simulink model "Proyecto1"  (R2023a)
settings: Solver=ode15s  StartTime=0.0  StopTime=12  MaxStep=0.0001  RelTol=1e-7  AbsTol=1e-9
libraries: fl_lib x22, nesl_utility x6, slpidlib x1
settings Model: Creator=ediel  LastModifiedBy=Chulis
settings SolverCC: AlgebraicLoopSolver=TrustRegion
settings DataIOCC: SaveOutput=off  SignalLogging=off  DSMLogging=off  ReturnWorkspaceOutputs=off  TimeSaveName=t
settings DebuggingCC: AlgebraicLoopMsg=none  ArtificialAlgebraicLoopMsg=none  MaxConsecutiveZCsMsg=none  UnconnectedInputMsg=warning  UnconnectedOutputMsg=warning  UnconnectedLineMsg=warning  ModelReferenceExtraNoncontSigs=none  OperatingPointInterfaceChecksumMismatchMsg=none
settings ModelReferenceCC: EnableRefExpFcnMdlSchedulingChecks=on
settings RTWCC: DLArmComputeVersion=19.05

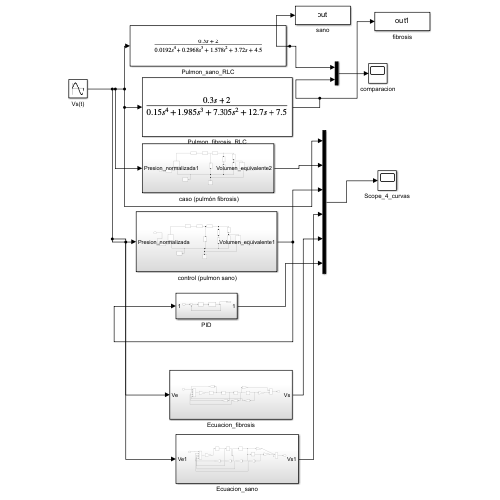
[thumbnail: Simulink's stored preview of the top-level diagram]
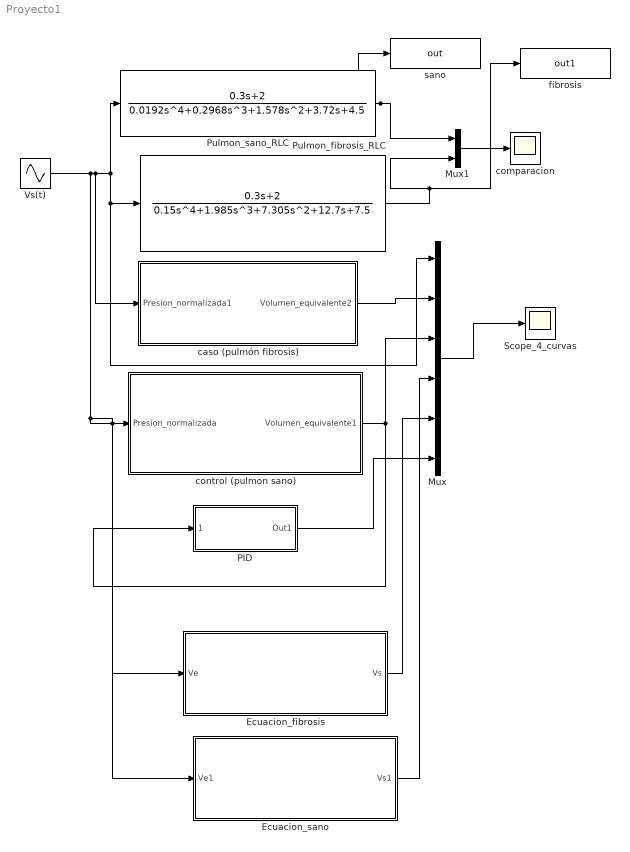
== system Proyecto1 ==
  " caso (pulmón fibrosis)" : Subsystem
  " control (pulmon sano)" : Subsystem
  Ecuacion_fibrosis : Subsystem
  Ecuacion_sano : Subsystem
  Mux : Mux  Inputs=6
  Mux1 : Mux  Inputs=2
  PID : Subsystem
  Pulmon_fibrosis_RLC : TransferFcn  Numerator=[0.3 2]  Denominator=[0.15,1.985,7.305,12.7,7.5]
  Pulmon_sano_RLC : TransferFcn  Numerator=[0.3 2]  Denominator=[0.0192,0.2968,1.578,3.72,4.5]
  Scope_4_curvas : Scope
  Vs(t) : Sin  Amplitude=0.5  Bias=0.5  Frequency=pi/2  Phase=-pi/2  SampleTime=0
  comparacion : Scope
  fibrosis : ToWorkspace  VariableName=out1  SaveFormat=Timeseries  SampleTime=-1
  sano : ToWorkspace  VariableName=out  SaveFormat=Timeseries  SampleTime=-1
  wires:
  Vs(t)/1 -> Ecuacion_sano/1(Ve1), Ecuacion_fibrosis/1(Ve), " control (pulmon sano)"/1(Presion_normalizada), Mux/1, Pulmon_fibrosis_RLC/1, Pulmon_sano_RLC/1, " caso (pulmón fibrosis)"/1(Presion_normalizada1)
  Pulmon_fibrosis_RLC/1 -> Mux1/2, fibrosis/1
  Pulmon_sano_RLC/1 -> Mux1/1, sano/1
  Mux/1 -> Scope_4_curvas/1
  " control (pulmon sano)"/1(Volumen_equivalente1) -> PID/1(1), Mux/3
  Mux1/1 -> comparacion/1
  " caso (pulmón fibrosis)"/1(Volumen_equivalente2) -> Mux/2
  PID/1(Out1) -> Mux/6
  Ecuacion_fibrosis/1(Vs) -> Mux/5
  Ecuacion_sano/1(Vs1) -> Mux/4

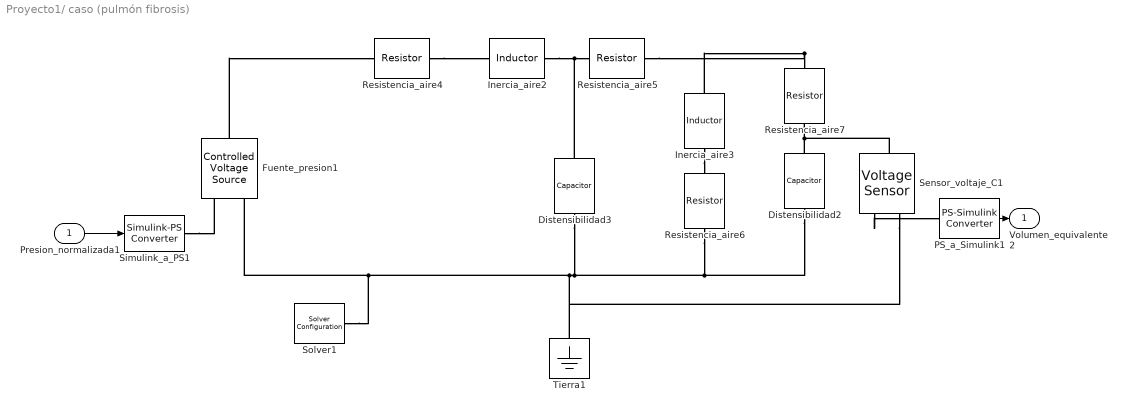
== system Proyecto1/ caso (pulmón fibrosis) ==
  Presion_normalizada1 : Inport
  Distensibilidad2 : fl_lib/Electrical/Electrical Elements/Capacitor  c=0.4 F  r=1e-6 Ohm  g=0 1/Ohm  i_specify=off  i_priority=None  i=0 A  i_nominal_specify=off  i_nominal_unit=A  i_nominal_value=1  v_specify=off  v_priority=None  v=0 V  v_nominal_specify=off  v_nominal_unit=V  v_nominal_value=1  vc_specify=off  vc_priority=High  vc=0 V  vc_nominal_specify=off  vc_nominal_unit=V  vc_nominal_value=1
  Distensibilidad3 : fl_lib/Electrical/Electrical Elements/Capacitor  c=0.5 F  r=1e-6 Ohm  g=0 1/Ohm  i_specify=off  i_priority=None  i=0 A  i_nominal_specify=off  i_nominal_unit=A  i_nominal_value=1  v_specify=off  v_priority=None  v=0 V  v_nominal_specify=off  v_nominal_unit=V  v_nominal_value=1  vc_specify=off  vc_priority=High  vc=0 V  vc_nominal_specify=off  vc_nominal_unit=V  vc_nominal_value=1
  Fuente_presion1 : fl_lib/Electrical/Electrical Sources/Controlled Voltage Source
  Inercia_aire2 : fl_lib/Electrical/Electrical Elements/Inductor  l=0.5 H  r=0.5 Ohm  g=1e-9 1/Ohm  i_specify=off  i_priority=None  i=0 A  i_nominal_specify=off  i_nominal_unit=A  i_nominal_value=1  v_specify=off  v_priority=None  v=0 V  v_nominal_specify=off  v_nominal_unit=V  v_nominal_value=1  i_L_specify=off  i_L_priority=High  i_L=0 A  i_L_nominal_specify=off  i_L_nominal_unit=A  i_L_nominal_value=1
  Inercia_aire3 : fl_lib/Electrical/Electrical Elements/Inductor  l=0.3 H  r=0 Ohm  g=1e-9 1/Ohm  i_specify=off  i_priority=None  i=0 A  i_nominal_specify=off  i_nominal_unit=A  i_nominal_value=1  v_specify=off  v_priority=None  v=0 V  v_nominal_specify=off  v_nominal_unit=V  v_nominal_value=1  i_L_specify=off  i_L_priority=High  i_L=0 A  i_L_nominal_specify=off  i_L_nominal_unit=A  i_L_nominal_value=1
  PS_a_Simulink1 : nesl_utility/PS-Simulink Converter  PhysicalDomain=network_engine_domain  SubClassName=ps_output  LeftPortType=input  RightPortType=output  PseudoPeriodic=off  Frequencies=[]  VectorFormat=1-D array  Unit=V  AffineConversion=off
  Resistencia_aire4 : fl_lib/Electrical/Electrical Elements/Resistor  R=1 Ohm  i_specify=off  i_priority=None  i=0 A  i_nominal_specify=off  i_nominal_unit=A  i_nominal_value=1  v_specify=off  v_priority=None  v=0 V  v_nominal_specify=off  v_nominal_unit=V  v_nominal_value=1
  Resistencia_aire5 : fl_lib/Electrical/Electrical Elements/Resistor  R=4 Ohm  i_specify=off  i_priority=None  i=0 A  i_nominal_specify=off  i_nominal_unit=A  i_nominal_value=1  v_specify=off  v_priority=None  v=0 V  v_nominal_specify=off  v_nominal_unit=V  v_nominal_value=1
  Resistencia_aire6 : fl_lib/Electrical/Electrical Elements/Resistor  R=2 Ohm  i_specify=off  i_priority=None  i=0 A  i_nominal_specify=off  i_nominal_unit=A  i_nominal_value=1  v_specify=off  v_priority=None  v=0 V  v_nominal_specify=off  v_nominal_unit=V  v_nominal_value=1
  Resistencia_aire7 : fl_lib/Electrical/Electrical Elements/Resistor  R=1 Ohm  i_specify=off  i_priority=None  i=0 A  i_nominal_specify=off  i_nominal_unit=A  i_nominal_value=1  v_specify=off  v_priority=None  v=0 V  v_nominal_specify=off  v_nominal_unit=V  v_nominal_value=1
  Sensor_voltaje_C1 : fl_lib/Electrical/Electrical Sensors/Voltage Sensor
  Simulink_a_PS1 : nesl_utility/Simulink-PS Converter  PhysicalDomain=network_engine_domain  SubClassName=ps_input  LeftPortType=input  RightPortType=output  PseudoPeriodic=off  Frequencies=[]  NoiseDistribution=none  NoiseParameters=[]  Unit=V  AffineConversion=off  FilteringAndDerivatives=provide  SimscapeFilterOrder=1  InputFilterTimeConstant=0.001  UdotUserProvided=0
  Solver1 : nesl_utility/Solver Configuration  PhysicalDomain=network_engine_domain  SubClassName=solver  LeftPortType=input  RightPortType=generic  Tones=[]  Harmonics=[]  SimulateNoise=off  Profile=off  UseLocalSampling=off  EnableSwitchedLinearOptims=on  FrequencyDomain=off  UseCCode=off  RelTol=0.001  AbsTol=1e-06  MinStep=1e-09  ToWorkspace=off  RevertToSquareIcSolve=off  NumHomotopyIterations=100  PhasorMode=off  PhasorModeNumHarmonics=1  ConsistencySolver=NEWTON_FTOL  IndexReductionMethod=DerivativeReplacement  DoDC=off  ResidualTolerance=1e-09  ConsistencyTolSource=GLOBAL  ConsistencyAbsTol=0.001  ConsistencyRelTol=0.001  ConsistencyTolFactor=0.001  UseLocalSolver=off  LocalSolverChoice=NE_BACKWARD_EULER_ADVANCER  ResolveIndetEquations=on  FunctionEvalNumThread=1  LocalSolverSampleTime=0.001  DoFixedCost=off  MaxNonlinIter=3  MaxModeIter=2  ComputeImpulses=off  ImpulseIterations=2  LinearAlgebra=auto  LinearAlgebraNumThread=0  EquationFormulation=NE_TIME_EF  DelaysMemoryBudget=1024  AutomaticFiltering=on  FilteringTimeConstant=0.001  PartitionStorageMethod=AS_NEEDED  PartitionMemoryBudget=1024  PartitionMethod=ROBUST
  Tierra1 : fl_lib/Electrical/Electrical Elements/Electrical Reference
  Volumen_equivalente2 : Outport
  wires:
  PS_a_Simulink1/1 -> Volumen_equivalente2/1
  Presion_normalizada1/1 -> Simulink_a_PS1/1
  connections:
  Resistencia_aire5/LConn1 -- Distensibilidad3/LConn1 -- Inercia_aire2/RConn1
  Resistencia_aire7/LConn1 -- Resistencia_aire5/RConn1 -- Inercia_aire3/LConn1
  Resistencia_aire6/RConn1 -- Sensor_voltaje_C1/RConn2 -- Tierra1/LConn1 -- Solver1/RConn1 -- Fuente_presion1/RConn2 -- Distensibilidad3/RConn1 -- Distensibilidad2/RConn1
  Fuente_presion1/LConn1 -- Resistencia_aire4/LConn1
  Resistencia_aire4/RConn1 -- Inercia_aire2/LConn1
  Inercia_aire3/RConn1 -- Resistencia_aire6/LConn1
  Distensibilidad2/LConn1 -- Sensor_voltaje_C1/LConn1 -- Resistencia_aire7/RConn1
  Simulink_a_PS1/RConn1 -- Fuente_presion1/RConn1
  Sensor_voltaje_C1/RConn1 -- PS_a_Simulink1/LConn1

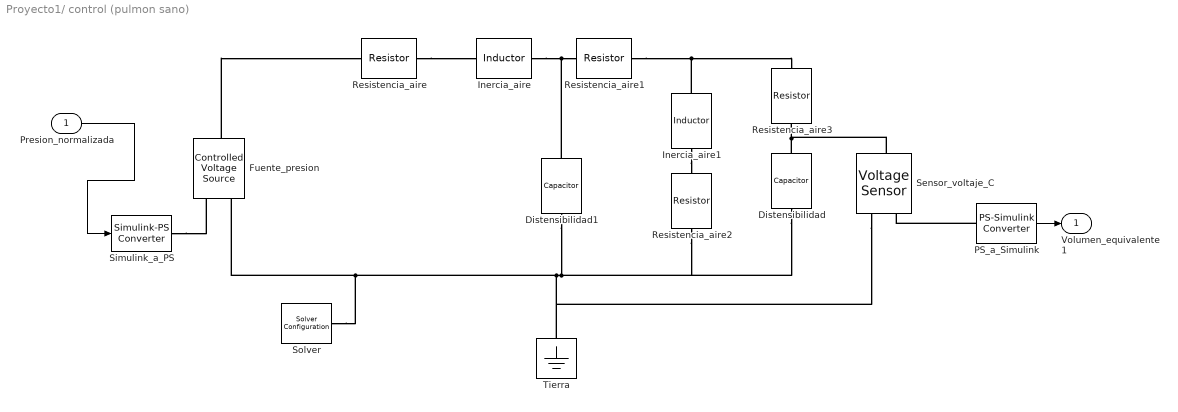
== system Proyecto1/ control (pulmon sano) ==
  Presion_normalizada : Inport
  Distensibilidad : fl_lib/Electrical/Electrical Elements/Capacitor  c=0.16 F  r=1e-6 Ohm  g=0 1/Ohm  i_specify=off  i_priority=None  i=0 A  i_nominal_specify=off  i_nominal_unit=A  i_nominal_value=1  v_specify=off  v_priority=None  v=0 V  v_nominal_specify=off  v_nominal_unit=V  v_nominal_value=1  vc_specify=off  vc_priority=High  vc=0 V  vc_nominal_specify=off  vc_nominal_unit=V  vc_nominal_value=1
  Distensibilidad1 : fl_lib/Electrical/Electrical Elements/Capacitor  c=0.2 F  r=1e-6 Ohm  g=0 1/Ohm  i_specify=off  i_priority=None  i=0 A  i_nominal_specify=off  i_nominal_unit=A  i_nominal_value=1  v_specify=off  v_priority=None  v=0 V  v_nominal_specify=off  v_nominal_unit=V  v_nominal_value=1  vc_specify=off  vc_priority=High  vc=0 V  vc_nominal_specify=off  vc_nominal_unit=V  vc_nominal_value=1
  Fuente_presion : fl_lib/Electrical/Electrical Sources/Controlled Voltage Source
  Inercia_aire : fl_lib/Electrical/Electrical Elements/Inductor  l=1 H  r=0.5 Ohm  g=1e-9 1/Ohm  i_specify=off  i_priority=None  i=0 A  i_nominal_specify=off  i_nominal_unit=A  i_nominal_value=1  v_specify=off  v_priority=None  v=0 V  v_nominal_specify=off  v_nominal_unit=V  v_nominal_value=1  i_L_specify=off  i_L_priority=High  i_L=0 A  i_L_nominal_specify=off  i_L_nominal_unit=A  i_L_nominal_value=1
  Inercia_aire1 : fl_lib/Electrical/Electrical Elements/Inductor  l=0.3 H  r=0 Ohm  g=1e-9 1/Ohm  i_specify=off  i_priority=None  i=0 A  i_nominal_specify=off  i_nominal_unit=A  i_nominal_value=1  v_specify=off  v_priority=None  v=0 V  v_nominal_specify=off  v_nominal_unit=V  v_nominal_value=1  i_L_specify=off  i_L_priority=High  i_L=0 A  i_L_nominal_specify=off  i_L_nominal_unit=A  i_L_nominal_value=1
  PS_a_Simulink : nesl_utility/PS-Simulink Converter  PhysicalDomain=network_engine_domain  SubClassName=ps_output  LeftPortType=input  RightPortType=output  PseudoPeriodic=off  Frequencies=[]  VectorFormat=1-D array  Unit=V  AffineConversion=off
  Resistencia_aire : fl_lib/Electrical/Electrical Elements/Resistor  R=1 Ohm  i_specify=off  i_priority=None  i=0 A  i_nominal_specify=off  i_nominal_unit=A  i_nominal_value=1  v_specify=off  v_priority=None  v=0 V  v_nominal_specify=off  v_nominal_unit=V  v_nominal_value=1
  Resistencia_aire1 : fl_lib/Electrical/Electrical Elements/Resistor  R=1 Ohm  i_specify=off  i_priority=None  i=0 A  i_nominal_specify=off  i_nominal_unit=A  i_nominal_value=1  v_specify=off  v_priority=None  v=0 V  v_nominal_specify=off  v_nominal_unit=V  v_nominal_value=1
  Resistencia_aire2 : fl_lib/Electrical/Electrical Elements/Resistor  R=2 Ohm  i_specify=off  i_priority=None  i=0 A  i_nominal_specify=off  i_nominal_unit=A  i_nominal_value=1  v_specify=off  v_priority=None  v=0 V  v_nominal_specify=off  v_nominal_unit=V  v_nominal_value=1
  Resistencia_aire3 : fl_lib/Electrical/Electrical Elements/Resistor  R=1 Ohm  i_specify=off  i_priority=None  i=0 A  i_nominal_specify=off  i_nominal_unit=A  i_nominal_value=1  v_specify=off  v_priority=None  v=0 V  v_nominal_specify=off  v_nominal_unit=V  v_nominal_value=1
  Sensor_voltaje_C : fl_lib/Electrical/Electrical Sensors/Voltage Sensor
  Simulink_a_PS : nesl_utility/Simulink-PS Converter  PhysicalDomain=network_engine_domain  SubClassName=ps_input  LeftPortType=input  RightPortType=output  PseudoPeriodic=off  Frequencies=[]  NoiseDistribution=none  NoiseParameters=[]  Unit=V  AffineConversion=off  FilteringAndDerivatives=provide  SimscapeFilterOrder=1  InputFilterTimeConstant=0.001  UdotUserProvided=0
  Solver : nesl_utility/Solver Configuration  PhysicalDomain=network_engine_domain  SubClassName=solver  LeftPortType=input  RightPortType=generic  Tones=[]  Harmonics=[]  SimulateNoise=off  Profile=off  UseLocalSampling=off  EnableSwitchedLinearOptims=on  FrequencyDomain=off  UseCCode=off  RelTol=0.001  AbsTol=1e-06  MinStep=1e-09  ToWorkspace=off  RevertToSquareIcSolve=off  NumHomotopyIterations=100  PhasorMode=off  PhasorModeNumHarmonics=1  ConsistencySolver=NEWTON_FTOL  IndexReductionMethod=DerivativeReplacement  DoDC=off  ResidualTolerance=1e-09  ConsistencyTolSource=GLOBAL  ConsistencyAbsTol=0.001  ConsistencyRelTol=0.001  ConsistencyTolFactor=0.001  UseLocalSolver=off  LocalSolverChoice=NE_BACKWARD_EULER_ADVANCER  ResolveIndetEquations=on  FunctionEvalNumThread=1  LocalSolverSampleTime=0.001  DoFixedCost=off  MaxNonlinIter=3  MaxModeIter=2  ComputeImpulses=off  ImpulseIterations=2  LinearAlgebra=auto  LinearAlgebraNumThread=0  EquationFormulation=NE_TIME_EF  DelaysMemoryBudget=1024  AutomaticFiltering=on  FilteringTimeConstant=0.001  PartitionStorageMethod=AS_NEEDED  PartitionMemoryBudget=1024  PartitionMethod=ROBUST
  Tierra : fl_lib/Electrical/Electrical Elements/Electrical Reference
  Volumen_equivalente1 : Outport
  wires:
  Presion_normalizada/1 -> Simulink_a_PS/1
  PS_a_Simulink/1 -> Volumen_equivalente1/1
  connections:
  Solver/RConn1 -- Sensor_voltaje_C/RConn2 -- Tierra/LConn1 -- Distensibilidad/RConn1 -- Resistencia_aire2/RConn1 -- Distensibilidad1/RConn1 -- Fuente_presion/RConn2
  Resistencia_aire/RConn1 -- Inercia_aire/LConn1
  Fuente_presion/LConn1 -- Resistencia_aire/LConn1
  Simulink_a_PS/RConn1 -- Fuente_presion/RConn1
  Resistencia_aire1/LConn1 -- Inercia_aire/RConn1 -- Distensibilidad1/LConn1
  Inercia_aire1/RConn1 -- Resistencia_aire2/LConn1
  Inercia_aire1/LConn1 -- Resistencia_aire1/RConn1 -- Resistencia_aire3/LConn1
  Distensibilidad/LConn1 -- Sensor_voltaje_C/LConn1 -- Resistencia_aire3/RConn1
  PS_a_Simulink/LConn1 -- Sensor_voltaje_C/RConn1

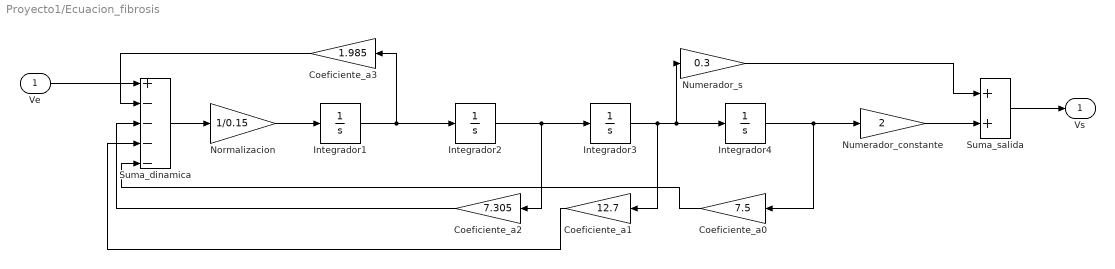
== system Proyecto1/Ecuacion_fibrosis ==
  Ve : Inport
  Coeficiente_a0 : Gain  Gain=7.5
  Coeficiente_a1 : Gain  Gain=12.7
  Coeficiente_a2 : Gain  Gain=7.305
  Coeficiente_a3 : Gain  Gain=1.985
  Integrador{1..4} (4 alike) : Integrator
  Normalizacion : Gain  Gain=1/0.15
  Numerador_constante : Gain  Gain=2
  Numerador_s : Gain  Gain=0.3
  Suma_dinamica : Sum  Inputs=+----
  Suma_salida : Sum
  Vs : Outport
  wires:
  Coeficiente_a3/1 -> Suma_dinamica/2
  Numerador_s/1 -> Suma_salida/1
  Numerador_constante/1 -> Suma_salida/2
  Integrador3/1 -> Integrador4/1, Numerador_s/1, Coeficiente_a1/1
  Integrador4/1 -> Coeficiente_a0/1, Numerador_constante/1
  Ve/1 -> Suma_dinamica/1
  Coeficiente_a1/1 -> Suma_dinamica/4
  Coeficiente_a2/1 -> Suma_dinamica/3
  Integrador2/1 -> Coeficiente_a2/1, Integrador3/1
  Coeficiente_a0/1 -> Suma_dinamica/5
  Suma_salida/1 -> Vs/1
  Suma_dinamica/1 -> Normalizacion/1
  Normalizacion/1 -> Integrador1/1
  Integrador1/1 -> Coeficiente_a3/1, Integrador2/1

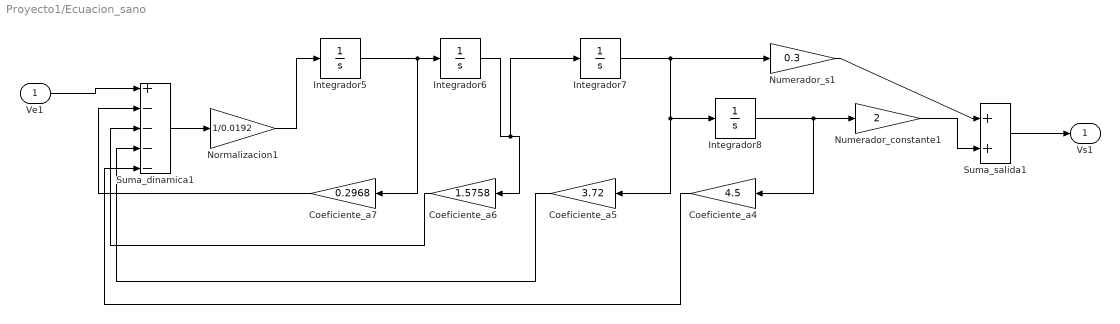
== system Proyecto1/Ecuacion_sano ==
  Ve1 : Inport
  Coeficiente_a4 : Gain  Gain=4.5
  Coeficiente_a5 : Gain  Gain=3.72
  Coeficiente_a6 : Gain  Gain=1.5758
  Coeficiente_a7 : Gain  Gain=0.2968
  Integrador{5..8} (4 alike) : Integrator
  Normalizacion1 : Gain  Gain=1/0.0192
  Numerador_constante1 : Gain  Gain=2
  Numerador_s1 : Gain  Gain=0.3
  Suma_dinamica1 : Sum  Inputs=+----
  Suma_salida1 : Sum
  Vs1 : Outport
  wires:
  Ve1/1 -> Suma_dinamica1/1
  Coeficiente_a7/1 -> Suma_dinamica1/2
  Integrador5/1 -> Coeficiente_a7/1, Integrador6/1
  Coeficiente_a5/1 -> Suma_dinamica1/4
  Integrador6/1 -> Integrador7/1, Coeficiente_a6/1
  Coeficiente_a6/1 -> Suma_dinamica1/3
  Numerador_constante1/1 -> Suma_salida1/2
  Integrador8/1 -> Coeficiente_a4/1, Numerador_constante1/1
  Integrador7/1 -> Coeficiente_a5/1, Integrador8/1, Numerador_s1/1
  Suma_salida1/1 -> Vs1/1
  Normalizacion1/1 -> Integrador5/1
  Suma_dinamica1/1 -> Normalizacion1/1
  Numerador_s1/1 -> Suma_salida1/1
  Coeficiente_a4/1 -> Suma_dinamica1/5

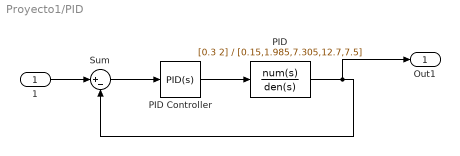
== system Proyecto1/PID ==
  1 : Inport
  "PID  " : TransferFcn  Numerator=[0.3 2]  Denominator=[0.15,1.985,7.305,12.7,7.5]
  PID Controller : slpidlib/PID Controller  Controller=PID  Form=Parallel  TimeDomain=Continuous-time  UseExternalTs=off  SampleTime=-1  IntegratorMethod=Forward Euler  FilterMethod=Forward Euler  ControllerParametersSource=internal  P=100000  I=0.0761  UseKiTs=off  D=99359  N=50108  UseFilter=on  TunerSelectOption=Frequency Response Based  InitialConditionSource=internal  InitialConditionForIntegrator=0  InitialConditionForFilter=0  DifferentiatorICPrevScaledInput=0  ExternalReset=none  TrackingMode=off  Kt=1  LimitOutput=off  SatLimitsSource=internal  UpperSaturationLimit=inf  LowerSaturationLimit=-inf  LinearizeAsGain=on  AntiWindupMode=none  Kb=1  LimitIntegrator=off  UpperIntegratorSaturationLimit=inf  LowerIntegratorSaturationLimit=-inf  POutMin=[]  POutMax=[]  IOutMin=[]  IOutMax=[]  DOutMin=[]  DOutMax=[]  NOutMin=[]  NOutMax=[]  SumOutMin=[]  SumOutMax=[]  SaturationOutMin=[]  SaturationOutMax=[]  PParamMin=[]  PParamMax=[]  IParamMin=[]  IParamMax=[]  DParamMin=[]  DParamMax=[]  NParamMin=[]  NParamMax=[]  KbParamMin=[]  KbParamMax=[]  KtParamMin=[]  KtParamMax=[]  KbOutMin=[]  KbOutMax=[]  KtOutMin=[]  KtOutMax=[]  IntegratorOutMin=[]  IntegratorOutMax=[]  FilterOutMin=[]  FilterOutMax=[]  SumI1OutMin=[]  SumI1OutMax=[]  SumI2OutMin=[]  SumI2OutMax=[]  SumI3OutMin=[]  SumI3OutMax=[]  SumI4OutMin=[]  SumI4OutMax=[]  SumDOutMin=[]  SumDOutMax=[]  DifferentiatorOutMin=[]  DifferentiatorOutMax=[]  FilterDiffOutCoefMin=[]  FilterDiffOutCoefMax=[]  ReciprocalOutMin=[]  ReciprocalOutMax=[]  SumDenOutMin=[]  SumDenOutMax=[]  SumNumOutMin=[]  SumNumOutMax=[]  DivideOutMin=[]  DivideOutMax=[]  UdiffTsProdOutMin=[]  UdiffTsProdOutMax=[]  NTsProdOutMin=[]  NTsProdOutMax=[]  UintegralTsProdOutMin=[]  UintegralTsProdOutMax=[]  UngainTsProdOutMin=[]  UngainTsProdOutMax=[]  ClampingZeroOutDataTypeStr=Inherit: Inherit via back propagation  ClampingZeroOutMin=[]  ClampingZeroOutMax=[]  FilterDenConstantOutDataTypeStr=Inherit: Inherit via back propagation  FilterDenConstantOutMin=[]  FilterDenConstantOutMax=[]  PCopyOutDataTypeStr=Inherit: Inherit via back propagation  PCopyOutMin=[]  PCopyOutMax=[]  NCopyOutDataTypeStr=Inherit: Inherit via back propagation  NCopyOutMin=[]  NCopyOutMax=[]  IntegratorContinuousStateAttributes=''  IntegratorStateMustResolveToSignalObject=off  IntegratorRTWStateStorageClass=Auto  FilterContinuousStateAttributes=''  FilterStateMustResolveToSignalObject=off  FilterRTWStateStorageClass=Auto  ParallelPVariant=InternalParameters  IdealPVariant=Disabled  IVariant=InternalParameters  DVariant=InternalParameters  IntegratorVariant=Continuous  SatVariant=Disabled  AWVariant=Passthrough  PCopyVariant=Disabled  TRVariant=Disabled  FdbkBlocksVariant=Forward  IdealPFdbkVariant=Disabled  SatFdbkVariant=Disabled  DerivativeFilterVariant=ContFilter  NVariant=InternalParameters  NCopyVariant=Disabled  FilterICVariant=InternalICsFilter  IntegratorICVariant=InternalICs  ExternalResetVariant=Disabled  TRSumVariant=Passthrough  SumFdbkVariant=Disabled  SumVariant=Sum_PID  TsampFilterVariant=InternalTs  TsampNgainVariant=Passthrough  TsampIntegralVariant=Disabled_SignalSpec  ExternalSaturationOutDataTypeStr=Inherit: Same as second input
  Sum : Sum  Inputs=|+-
  Out1 : Outport
  wires:
  PID Controller/1 -> "PID  "/1
  Sum/1 -> PID Controller/1
  "PID  "/1 -> Out1/1, Sum/2
  1/1 -> Sum/1
